simulink model "MotorCC_V2_R2024b"  (R2024b)
settings: Solver=VariableStepAuto  StartTime=0.0  StopTime=inf  RelTol=1e-3
undefined symbols (not defined in the file or in its folder): LF
libraries: instrumentseriallib x3
settings Model: PacingRate=0.010000  Creator=ignacioalvarado  LastModifiedBy=ignacioalvarado
settings OptimizationCC: ReuseModelBlockBuffer=off
settings RTWCC: GPUComputeCapability=3.5
settings ConfigComp: CovBoundaryAbsTol=1.0e-5

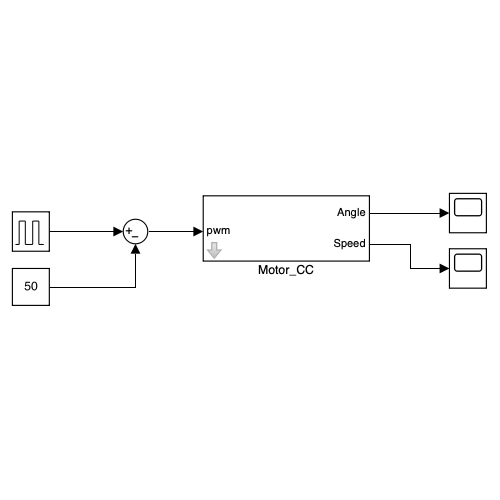
[thumbnail: Simulink's stored preview of the top-level diagram]
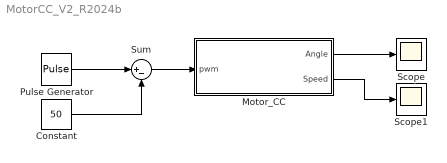
== system MotorCC_V2_R2024b ==
  Constant : Constant  Value=50
  Motor_CC : Subsystem  mask{PortName=/dev/cu.usbmodem23101}
      mask prompts: PortName "Arduino Port:"
      mask init:
      | % Obtener lista de puertos serie disponibles
      |     serialInfo = instrhwinfo('serial');
      |     availablePorts = serialInfo.AvailableSerialPorts;
      | 
      | % Si no hay puertos disponibles, establecer un mensaje predeterminado
      |     if isempty(availablePorts)
      |         availablePorts = {'No Ports Available'};
      |     end
      | 
      | % Obtener el objeto de la máscara
      |     maskObj = Simulink.Mask.get(gcb);
      |     portParam = maskObj.getParameter('PortName');
      | 
      | % Actualizar la lista desplegable con los puertos disponibles
      |     portParam.TypeOptions = availablePorts;
      | 
      | % Si el valor actual de 'PortName' no está en la lista, selecciona el primer puerto disponible
      |     currentPort = get_param(gcb, 'PortName');
      |     if ~ismember(currentPort, availablePorts)
      |         set_param(gcb, 'PortName', availablePorts{1});
      |     end
      |     assignin('base', 'PortName', get_param(gcb, 'PortName'));
      |     set_param([gcb, '/Serial Configuration'], 'Port', get_param(gcb, 'PortName'));
      |     set_param([gcb, '/Serial Send'], 'Port', get_param(gcb, 'PortName'));
      |     set_param([gcb, '/Serial Receive'], 'Port', get_param(gcb, 'PortName'));
      mask TypeOptions PortName: /dev/tty.debug-console | /dev/cu.debug-console | /dev/tty.wlan-debug | /dev/cu.wlan-debug | /dev/tty.Bluetooth-Incoming-Port | /dev/cu.Bluetooth-Incoming-Port | /dev/tty.cascos | /dev/cu.cascos | /dev/tty.GalaxyBudsLive76A9 | /dev/cu.GalaxyBudsLive76A9 | /dev/tty.usbmodem23101 | /dev/cu.usbmodem23101
  Pulse Generator : DiscretePulseGenerator  PulseType=Time based  Amplitude=50  Period=10  PulseWidth=50
  Scope : Scope
  Scope1 : Scope
  Sum : Sum  Inputs=|+-
  wires:
  Pulse Generator/1 -> Sum/1
  Constant/1 -> Sum/2
  Sum/1 -> Motor_CC/1(pwm)
  Motor_CC/1(Angle) -> Scope/1
  Motor_CC/2(Speed) -> Scope1/1

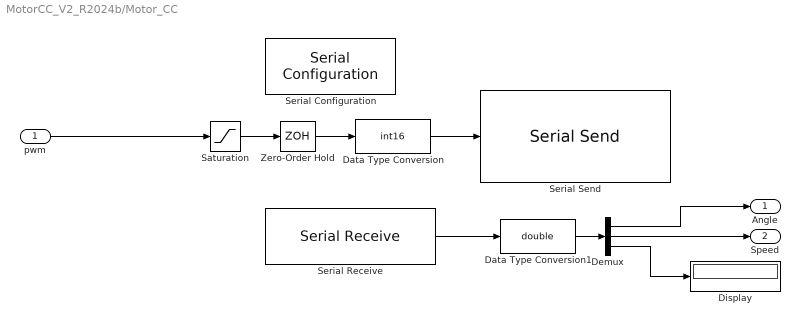
== system MotorCC_V2_R2024b/Motor_CC ==
  pwm : Inport
  Data Type Conversion : DataTypeConversion  OutDataTypeStr=int16  SaturateOnIntegerOverflow=off  RndMeth=Floor  LockScale=on
  Data Type Conversion1 : DataTypeConversion  OutDataTypeStr=double  SaturateOnIntegerOverflow=off  RndMeth=Floor
  Demux : Demux  Outputs=3
  Display : Display
  Saturation : Saturate  UpperLimit=255  LowerLimit=-255
  Serial Configuration : instrumentseriallib/Serial Configuration  Priority=-200000  PortSel=/dev/cu.usbmodem23101  Port=/dev/cu.usbmodem23101  ComPort=/dev/cu.usbmodem23101  BaudRate=115200  DataBits=8  Parity=none  StopBits=1  ByteOrder=little-endian  FlowControl=none  Timeout=10  SimulateUsing=Interpreted execution  BlockInModel=on  aMode=1
  Serial Receive : instrumentseriallib/Serial Receive  Priority=1  PortSel=/dev/cu.usbmodem23101  Port=/dev/cu.usbmodem23101  ComPort=/dev/cu.usbmodem23101  DataType=single  SaveDataType=uint8  ToggleHeader=on  Header='V'  ToggleDataSize=on  DataSize=[1 3]  ToggleTerminator=on  Terminator=LF ('\n')  CustomTerminator=[]  InputFormat=Row major  EnableBlockingMode=on  ActionDataUnavailable=Output last received value  ActionWhenDataUnavailable=Output last received value  CustomValue=0  SampleTime=0.01  SimulateUsing=Interpreted execution  BlockInModel=on  aMode=1
  Serial Send : instrumentseriallib/Serial Send  Priority=1  PortSel=/dev/cu.usbmodem23101  Port=/dev/cu.usbmodem23101  ComPort=/dev/cu.usbmodem23101  Header='A'  Terminator=LF ('\n')  CustomTerminator=[]  EnableBlockingMode=on  SimulateUsing=Interpreted execution  BlockInModel=on  aMode=1
  Zero-Order Hold : ZeroOrderHold  SampleTime=0.01
  Angle : Outport
  Speed : Outport  Port=2
  wires:
  Serial Receive/1 -> Data Type Conversion1/1
  Data Type Conversion/1 -> Serial Send/1
  pwm/1 -> Saturation/1
  Zero-Order Hold/1 -> Data Type Conversion/1
  Saturation/1 -> Zero-Order Hold/1
  Data Type Conversion1/1 -> Demux/1
  Demux/2 -> Speed/1
  Demux/1 -> Angle/1
  Demux/3 -> Display/1
